simulink model "r2_b8a4x128f_4gbe"  (R2012b)
settings: Solver=VariableStepDiscrete  SolverMode=SingleTasking  StartTime=0.0  StopTime=1  RelTol=1e-3
undefined symbols (not defined in the file): fft_stages, n_ants, n_bits_xengs
libraries: xbsIndex_r4 x21845, casper_library_misc x157, xbsReplacements_r4 x24, casper_library_communications x8, casper_library_delays x8, xps_library x5
(part 58 of 182)

== system r2_b8a4x128f_4gbe/sys3/vacc_tvg ==
  tvg_sel : Inport
  sync_in : Inport  Port=2
  data_in : Inport  Port=3
  valid_in : Inport  Port=4
  misci : Inport  Port=5
  Delay{,1..4} (5 alike) : xbsIndex_r4/Delay  rst=off  infoeditControl=Selection of Reset will increase slice count due to use of real FFs and instead of SRLs  en=off  latency=1  dbl_ovrd=off  reg_retiming=on  block_type=delay
      settings: xl_area=[0, 0, 0, 0, 0, 0, 0]
  Mux1 : xbsIndex_r4/Mux  inputs=2  en=off  latency=0  precision=Full  arith_type="Signed  (2's comp)"  n_bits=8  bin_pt=2  quantization=Truncate  overflow=Wrap  dbl_ovrd=off  block_type=mux
      settings: xl_area=[0, 0, 0, 0, 0, 0, 0]
  Mux2 : xbsIndex_r4/Mux  inputs=2  en=off  latency=0  precision=Full  arith_type="Signed  (2's comp)"  n_bits=8  bin_pt=2  quantization=Truncate  overflow=Wrap  dbl_ovrd=off  block_type=mux
      settings: xl_area=[0, 0, 0, 0, 0, 0, 0]
  Mux3 : xbsIndex_r4/Mux  inputs=2  en=off  latency=0  precision=Full  arith_type="Signed  (2's comp)"  n_bits=8  bin_pt=2  quantization=Truncate  overflow=Wrap  dbl_ovrd=off  block_type=mux
      settings: xl_area=[0, 0, 0, 0, 0, 0, 0]
  Slice : xbsIndex_r4/Slice  nbits=n_bits  boolean_output=off  mode=Lower Bit Location + Width  bit1=0  base1=MSB of Input  bit0=0  base0=LSB of Input  dbl_ovrd=off  block_type=slice
  Slice1 : xbsIndex_r4/Slice  nbits=1  boolean_output=on  mode=Lower Bit Location + Width  bit1=0  base1=MSB of Input  bit0=4  base0=LSB of Input  dbl_ovrd=off  block_type=slice
      settings: infoedit="Extracts a given range of bits from each input sample and presents it at the output.  The output type is ordinarily unsigned with binary point at zero, but can be Boolean when the slice is one bit wide.<P><P>Hardware notes: In hardware this block costs nothing."  block_version=10.1.3
  Slice2 : xbsIndex_r4/Slice  nbits=1  boolean_output=on  mode=Lower Bit Location + Width  bit1=0  base1=MSB of Input  bit0=0  base0=LSB of Input  dbl_ovrd=off  block_type=slice
      settings: infoedit="Extracts a given range of bits from each input sample and presents it at the output.  The output type is ordinarily unsigned with binary point at zero, but can be Boolean when the slice is one bit wide.<P><P>Hardware notes: In hardware this block costs nothing."  block_version=10.1.3
  Slice3 : xbsIndex_r4/Slice  nbits=1  boolean_output=on  mode=Lower Bit Location + Width  bit1=0  base1=MSB of Input  bit0=3  base0=LSB of Input  dbl_ovrd=off  block_type=slice
      settings: infoedit="Extracts a given range of bits from each input sample and presents it at the output.  The output type is ordinarily unsigned with binary point at zero, but can be Boolean when the slice is one bit wide.<P><P>Hardware notes: In hardware this block costs nothing."  block_version=10.1.3
  Slice4 : xbsIndex_r4/Slice  nbits=1  boolean_output=on  mode=Lower Bit Location + Width  bit1=0  base1=MSB of Input  bit0=2  base0=LSB of Input  dbl_ovrd=off  block_type=slice
      settings: infoedit="Extracts a given range of bits from each input sample and presents it at the output.  The output type is ordinarily unsigned with binary point at zero, but can be Boolean when the slice is one bit wide.<P><P>Hardware notes: In hardware this block costs nothing."  block_version=10.1.3
  Slice5 : xbsIndex_r4/Slice  nbits=1  boolean_output=on  mode=Lower Bit Location + Width  bit1=0  base1=MSB of Input  bit0=1  base0=LSB of Input  dbl_ovrd=off  block_type=slice
      settings: infoedit="Extracts a given range of bits from each input sample and presents it at the output.  The output type is ordinarily unsigned with binary point at zero, but can be Boolean when the slice is one bit wide.<P><P>Hardware notes: In hardware this block costs nothing."  block_version=10.1.3
  Slice6 : xbsIndex_r4/Slice  nbits=1  boolean_output=on  mode=Lower Bit Location + Width  bit1=0  base1=MSB of Input  bit0=0  base0=LSB of Input  dbl_ovrd=off  block_type=slice
      settings: infoedit="Extracts a given range of bits from each input sample and presents it at the output.  The output type is ordinarily unsigned with binary point at zero, but can be Boolean when the slice is one bit wide.<P><P>Hardware notes: In hardware this block costs nothing."  block_version=10.1.3
  Slice7 : xbsIndex_r4/Slice  nbits=1  boolean_output=on  mode=Lower Bit Location + Width  bit1=0  base1=MSB of Input  bit0=5  base0=LSB of Input  dbl_ovrd=off  block_type=slice
      settings: infoedit="Extracts a given range of bits from each input sample and presents it at the output.  The output type is ordinarily unsigned with binary point at zero, but can be Boolean when the slice is one bit wide.<P><P>Hardware notes: In hardware this block costs nothing."  block_version=10.1.3
  Slice8 : xbsIndex_r4/Slice  nbits=n_bits  boolean_output=off  mode=Lower Bit Location + Width  bit1=0  base1=MSB of Input  bit0=0  base0=LSB of Input  dbl_ovrd=off  block_type=slice
  Terminator{1..5} (5 alike) : Terminator
  bus_replicate : Subsystem  AncestorBlock=casper_library_bus/bus_replicate  mask(bus_replicate){replication=n_inputs, latency=0, misc=off, implementation=core}
      mask prompts: replication "replication factor"; misc "misc support"; implementation "delay implementation"
      mask help: Output bus formed by replicating input bus a number of times
      mask init:
      | bus_replicate_init(gcb, ...
      |     'replication', replication, ...
      |     'latency', latency, ...
      |     'implementation', implementation, ...
      |     'misc', misc);
      mask TypeOptions implementation: core | behavioral
  bus_replicate1 : Subsystem  AncestorBlock=casper_library_bus/bus_replicate  mask(bus_replicate){replication=n_inputs, latency=0, misc=off, implementation=core}
      mask prompts: replication "replication factor"; misc "misc support"; implementation "delay implementation"
      mask help: Output bus formed by replicating input bus a number of times
      mask init:
      | bus_replicate_init(gcb, ...
      |     'replication', replication, ...
      |     'latency', latency, ...
      |     'implementation', implementation, ...
      |     'misc', misc);
      mask TypeOptions implementation: core | behavioral
  edge_detect : Subsystem  AncestorBlock=casper_library_misc/edge_detect  mask(edge_detect){edge=Rising, polarity=Active High, x_in=[0 0.08 0.08 0.16 0.16 0.24 0.24 0.32 0.32 0.4], y_in=[-1 -1  1  1  1  1  1  1  1  1], x_out=[0.6 0.68 0.68 0.76 0.76 0.84 0.84 0.92 0.92 1], y_out=[-1 -1  1  1 -1 -1 -1 -1 -1 -1]}
      mask prompts: edge "Edge Type"; polarity "Output Polarity"; x_in "Input X Positions"; y_in "Input Y Positions"; x_out "Output X Positions"; y_out "Output Y Positions"
      mask help: Output is active for one-cycle after each edge of the specified type (i.e. rising, falling or both).
      mask init: same as r2_b8a4x128f_4gbe/edge_detect
      settings: AttributesFormatString=|
      | rising edges
      | active high
      mask Help: Output is active for one-cycle after each edge of the specified type (i.e. rising, falling, or both).  Latency is zero.
      mask TypeOptions edge: Rising | Falling | Both
      mask TypeOptions polarity: Active High | Active Low
      mask Display:
      | plot(x_in_num,0.5+y_in_num*0.2);
      | plot(x_out_num,0.5+y_out_num*0.2);
  generate_pulses : Subsystem
  group_period : Subsystem  Tag=xps:sw_reg  AncestorBlock=xps_library/software register  mask(swreg){mode=one value, io_dir=From Processor, io_delay=0, sample_period=1, names=reg, bitwidths=32, arith_types=0, bin_pts=0, show_format=off}
      mask prompts: io_dir "I/O direction"; io_delay "I/O delay"; sample_period "Sample period"; names "Name:"; bitwidths "Bitwidth:"; arith_types "Type (ufix=0, fix=1, bool=2):"; bin_pts "Binary pt:"; show_format "Print format string?"
      mask init:
      | swreg_init(gcb)
      settings: AttributesFormatString=1input
      mask TypeOptions mode: one value | fields of equal size | fields of arbitrary size
      mask Callback mode: swreg_cb(gcb);
      mask TypeOptions io_dir: To Processor | From Processor
      mask Callback io_dir:
      | mask_enables = get_param(gcb, 'MaskEnables');
      | mask_names = get_param(gcb, 'MaskNames');
      | if strcmp(get_param(gcb, 'io_dir'), 'To Processor'),
      |     mask_enables{ismember(mask_names, 'sample_period')} = 'off';
      | else
      |     mask_enables{ismember(mask_names, 'sample_period')} = 'on';
      | end
      | set_param(gcb, 'MaskEnables', mask_enables);
      mask Callback bitwidths:
      | blk = gcb;
      | mode = get_param(blk, 'mode');
      | current_widths = eval(get_param(blk, 'bitwidths'));
      | if (strcmp(mode, 'one value') || strcmp(mode, 'fields of equal size')) && (length(current_widths) > 1),
      |     error('Only one width may be specified for this mode.');
      | elseif strcmp(mode, 'fields of arbitrary size')
      |     current_names = textscan(strtrim(strrep(strrep(get_param(blk, 'names'), ']', ''), '[', '')), '%s');
      |     current_names = current_names{1};
      |     numios = length(current_names);
      |     if length(current_widths) ~= numios,
      |         error('%d field names specified, but %d widths?', numios, length(current_widths));
      |     end
      | end
      | total_width = 0;
      | for ctr = 1 : length(current_widths),
      |     total_width = total_width + current_widths(ctr);
      | end
      | if total_width > 32,
      |     error('Total width must be 32 or less, set to %d.', total_width);
      | end
      mask Callback arith_types:
      | blk = gcb;
      | mode = get_param(blk, 'mode');
      | current_types = eval(get_param(blk, 'arith_types'));
      | numios = length(current_types);
      | if (strcmp(mode, 'one value') || strcmp(mode, 'fields of equal size')) && (length(current_types) > 1),
      |     error('Only one type may be specified for this mode.');
      | elseif strcmp(mode, 'fields of arbitrary size')
      |     current_names = textscan(strtrim(strrep(strrep(get_param(blk, 'names'), ']', ''), '[', '')), '%s');
      |     current_names = current_names{1};
      |     numios = length(current_names);
      |     if length(current_types) ~= numios,
      |         error('%d field names specified, but %d types?', numios, length(current_types));
      |     end
      | end
      | problem = 0;
      | for ctr = 1 : numios,
      |     t = current_types(ctr);
      |     if (t < 0) || (t > 2),
      |         problem = t;
      |         ctr = numios + 1;
      |     end
      | end
      | if problem ~= 0,
      |     error('Type cannot be %i, must be 0, 1 or 2.', problem);
      | end
      mask Callback bin_pts:
      | blk = gcb;
      | mode = get_param(blk, 'mode');
      | current_bins = eval(get_param(blk, 'bin_pts'));
      | if (strcmp(mode, 'one value') || strcmp(mode, 'fields of equal size')) && (length(current_bins) > 1),
      |     error('Only one binary pt may be specified for this mode.');
      | elseif strcmp(mode, 'fields of arbitrary size')
      |     current_names = textscan(strtrim(strrep(strrep(get_param(blk, 'names'), ']', ''), '[', '')), '%s');
      |     current_names = current_names{1};
      |     numios = length(current_names);
      |     if length(current_bins) ~= numios,
      |         error('%d field names specified, but %d binary pts?', numios, length(current_bins));
      |     end
      | end
  ins_counter : Subsystem  mask{vec_len=len/n_inputs, n_inputs=n_inputs, n_bits=n_bits}
      mask prompts: vec_len "Vector Length?"; n_inputs "Simultaneous inputs"; n_bits "Data width"
      mask init:
      | fmtstr = sprintf('Vector Length: %d', vec_len);
      | set_param(gcb, 'AttributesFormatString', fmtstr);
      settings: AttributesFormatString=Vector Length: 9216
  ins_vect_loc : Subsystem  Tag=xps:sw_reg  AncestorBlock=xps_library/software register  mask(swreg){mode=one value, io_dir=From Processor, io_delay=0, sample_period=1, names=reg, bitwidths=32, arith_types=0, bin_pts=0, show_format=off}
      mask prompts: io_dir "I/O direction"; io_delay "I/O delay"; sample_period "Sample period"; names "Name:"; bitwidths "Bitwidth:"; arith_types "Type (ufix=0, fix=1, bool=2):"; bin_pts "Binary pt:"; show_format "Print format string?"
      mask init:
      | swreg_init(gcb)
      settings: AttributesFormatString=1input
      mask TypeOptions mode: one value | fields of equal size | fields of arbitrary size
      mask Callback mode: swreg_cb(gcb);
      mask TypeOptions io_dir: To Processor | From Processor
      mask Callback io_dir:
      | mask_enables = get_param(gcb, 'MaskEnables');
      | mask_names = get_param(gcb, 'MaskNames');
      | if strcmp(get_param(gcb, 'io_dir'), 'To Processor'),
      |     mask_enables{ismember(mask_names, 'sample_period')} = 'off';
      | else
      |     mask_enables{ismember(mask_names, 'sample_period')} = 'on';
      | end
      | set_param(gcb, 'MaskEnables', mask_enables);
      mask Callback bitwidths:
      | blk = gcb;
      | mode = get_param(blk, 'mode');
      | current_widths = eval(get_param(blk, 'bitwidths'));
      | if (strcmp(mode, 'one value') || strcmp(mode, 'fields of equal size')) && (length(current_widths) > 1),
      |     error('Only one width may be specified for this mode.');
      | elseif strcmp(mode, 'fields of arbitrary size')
      |     current_names = textscan(strtrim(strrep(strrep(get_param(blk, 'names'), ']', ''), '[', '')), '%s');
      |     current_names = current_names{1};
      |     numios = length(current_names);
      |     if length(current_widths) ~= numios,
      |         error('%d field names specified, but %d widths?', numios, length(current_widths));
      |     end
      | end
      | total_width = 0;
      | for ctr = 1 : length(current_widths),
      |     total_width = total_width + current_widths(ctr);
      | end
      | if total_width > 32,
      |     error('Total width must be 32 or less, set to %d.', total_width);
      | end
      mask Callback arith_types:
      | blk = gcb;
      | mode = get_param(blk, 'mode');
      | current_types = eval(get_param(blk, 'arith_types'));
      | numios = length(current_types);
      | if (strcmp(mode, 'one value') || strcmp(mode, 'fields of equal size')) && (length(current_types) > 1),
      |     error('Only one type may be specified for this mode.');
      | elseif strcmp(mode, 'fields of arbitrary size')
      |     current_names = textscan(strtrim(strrep(strrep(get_param(blk, 'names'), ']', ''), '[', '')), '%s');
      |     current_names = current_names{1};
      |     numios = length(current_names);
      |     if length(current_types) ~= numios,
      |         error('%d field names specified, but %d types?', numios, length(current_types));
      |     end
      | end
      | problem = 0;
      | for ctr = 1 : numios,
      |     t = current_types(ctr);
      |     if (t < 0) || (t > 2),
      |         problem = t;
      |         ctr = numios + 1;
      |     end
      | end
      | if problem ~= 0,
      |     error('Type cannot be %i, must be 0, 1 or 2.', problem);
      | end
      mask Callback bin_pts:
      | blk = gcb;
      | mode = get_param(blk, 'mode');
      | current_bins = eval(get_param(blk, 'bin_pts'));
      | if (strcmp(mode, 'one value') || strcmp(mode, 'fields of equal size')) && (length(current_bins) > 1),
      |     error('Only one binary pt may be specified for this mode.');
      | elseif strcmp(mode, 'fields of arbitrary size')
      |     current_names = textscan(strtrim(strrep(strrep(get_param(blk, 'names'), ']', ''), '[', '')), '%s');
      |     current_names = current_names{1};
      |     numios = length(current_names);
      |     if length(current_bins) ~= numios,
      |         error('%d field names specified, but %d binary pts?', numios, length(current_bins));
      |     end
      | end
  ins_vect_val : Subsystem  Tag=xps:sw_reg  AncestorBlock=xps_library/software register  mask(swreg){mode=one value, io_dir=From Processor, io_delay=0, sample_period=1, names=reg, bitwidths=32, arith_types=0, bin_pts=0, show_format=off}
      mask prompts: io_dir "I/O direction"; io_delay "I/O delay"; sample_period "Sample period"; names "Name:"; bitwidths "Bitwidth:"; arith_types "Type (ufix=0, fix=1, bool=2):"; bin_pts "Binary pt:"; show_format "Print format string?"
      mask init:
      | swreg_init(gcb)
      settings: AttributesFormatString=1input
      mask TypeOptions mode: one value | fields of equal size | fields of arbitrary size
      mask Callback mode: swreg_cb(gcb);
      mask TypeOptions io_dir: To Processor | From Processor
      mask Callback io_dir:
      | mask_enables = get_param(gcb, 'MaskEnables');
      | mask_names = get_param(gcb, 'MaskNames');
      | if strcmp(get_param(gcb, 'io_dir'), 'To Processor'),
      |     mask_enables{ismember(mask_names, 'sample_period')} = 'off';
      | else
      |     mask_enables{ismember(mask_names, 'sample_period')} = 'on';
      | end
      | set_param(gcb, 'MaskEnables', mask_enables);
      mask Callback bitwidths:
      | blk = gcb;
      | mode = get_param(blk, 'mode');
      | current_widths = eval(get_param(blk, 'bitwidths'));
      | if (strcmp(mode, 'one value') || strcmp(mode, 'fields of equal size')) && (length(current_widths) > 1),
      |     error('Only one width may be specified for this mode.');
      | elseif strcmp(mode, 'fields of arbitrary size')
      |     current_names = textscan(strtrim(strrep(strrep(get_param(blk, 'names'), ']', ''), '[', '')), '%s');
      |     current_names = current_names{1};
      |     numios = length(current_names);
      |     if length(current_widths) ~= numios,
      |         error('%d field names specified, but %d widths?', numios, length(current_widths));
      |     end
      | end
      | total_width = 0;
      | for ctr = 1 : length(current_widths),
      |     total_width = total_width + current_widths(ctr);
      | end
      | if total_width > 32,
      |     error('Total width must be 32 or less, set to %d.', total_width);
      | end
      mask Callback arith_types:
      | blk = gcb;
      | mode = get_param(blk, 'mode');
      | current_types = eval(get_param(blk, 'arith_types'));
      | numios = length(current_types);
      | if (strcmp(mode, 'one value') || strcmp(mode, 'fields of equal size')) && (length(current_types) > 1),
      |     error('Only one type may be specified for this mode.');
      | elseif strcmp(mode, 'fields of arbitrary size')
      |     current_names = textscan(strtrim(strrep(strrep(get_param(blk, 'names'), ']', ''), '[', '')), '%s');
      |     current_names = current_names{1};
      |     numios = length(current_names);
      |     if length(current_types) ~= numios,
      |         error('%d field names specified, but %d types?', numios, length(current_types));
      |     end
      | end
      | problem = 0;
      | for ctr = 1 : numios,
      |     t = current_types(ctr);
      |     if (t < 0) || (t > 2),
      |         problem = t;
      |         ctr = numios + 1;
      |     end
      | end
      | if problem ~= 0,
      |     error('Type cannot be %i, must be 0, 1 or 2.', problem);
      | end
      mask Callback bin_pts:
      | blk = gcb;
      | mode = get_param(blk, 'mode');
      | current_bins = eval(get_param(blk, 'bin_pts'));
      | if (strcmp(mode, 'one value') || strcmp(mode, 'fields of equal size')) && (length(current_bins) > 1),
      |     error('Only one binary pt may be specified for this mode.');
      | elseif strcmp(mode, 'fields of arbitrary size')
      |     current_names = textscan(strtrim(strrep(strrep(get_param(blk, 'names'), ']', ''), '[', '')), '%s');
      |     current_names = current_names{1};
      |     numios = length(current_names);
      |     if length(current_bins) ~= numios,
      |         error('%d field names specified, but %d binary pts?', numios, length(current_bins));
      |     end
      | end
  ins_vector : Subsystem  mask{num_vectors=len/n_inputs}
      mask prompts: num_vectors "number of vectors"
      mask init:
      | fmtstr = sprintf('Vector Length: %d', num_vectors);
      | set_param(gcb, 'AttributesFormatString', fmtstr);
      settings: AttributesFormatString=Vector Length: 9216
  master_reset_sim1 : Constant  Value=0
  master_reset_sim10 : Constant  Value=1000
  master_reset_sim11 : Constant  Value=127
  master_reset_sim4 : Constant  Value=0
  master_reset_sim7 : Constant  Value=512000
  master_reset_sim8 : Constant
  master_reset_sim9 : Constant  Value=3
  n_per_group : Subsystem  Tag=xps:sw_reg  AncestorBlock=xps_library/software register  mask(swreg){mode=one value, io_dir=From Processor, io_delay=0, sample_period=1, names=reg, bitwidths=32, arith_types=0, bin_pts=0, show_format=off}
      mask prompts: io_dir "I/O direction"; io_delay "I/O delay"; sample_period "Sample period"; names "Name:"; bitwidths "Bitwidth:"; arith_types "Type (ufix=0, fix=1, bool=2):"; bin_pts "Binary pt:"; show_format "Print format string?"
      mask init:
      | swreg_init(gcb)
      settings: AttributesFormatString=1input
      mask TypeOptions mode: one value | fields of equal size | fields of arbitrary size
      mask Callback mode: swreg_cb(gcb);
      mask TypeOptions io_dir: To Processor | From Processor
      mask Callback io_dir:
      | mask_enables = get_param(gcb, 'MaskEnables');
      | mask_names = get_param(gcb, 'MaskNames');
      | if strcmp(get_param(gcb, 'io_dir'), 'To Processor'),
      |     mask_enables{ismember(mask_names, 'sample_period')} = 'off';
      | else
      |     mask_enables{ismember(mask_names, 'sample_period')} = 'on';
      | end
      | set_param(gcb, 'MaskEnables', mask_enables);
      mask Callback bitwidths:
      | blk = gcb;
      | mode = get_param(blk, 'mode');
      | current_widths = eval(get_param(blk, 'bitwidths'));
      | if (strcmp(mode, 'one value') || strcmp(mode, 'fields of equal size')) && (length(current_widths) > 1),
      |     error('Only one width may be specified for this mode.');
      | elseif strcmp(mode, 'fields of arbitrary size')
      |     current_names = textscan(strtrim(strrep(strrep(get_param(blk, 'names'), ']', ''), '[', '')), '%s');
      |     current_names = current_names{1};
      |     numios = length(current_names);
      |     if length(current_widths) ~= numios,
      |         error('%d field names specified, but %d widths?', numios, length(current_widths));
      |     end
      | end
      | total_width = 0;
      | for ctr = 1 : length(current_widths),
      |     total_width = total_width + current_widths(ctr);
      | end
      | if total_width > 32,
      |     error('Total width must be 32 or less, set to %d.', total_width);
      | end
      mask Callback arith_types:
      | blk = gcb;
      | mode = get_param(blk, 'mode');
      | current_types = eval(get_param(blk, 'arith_types'));
      | numios = length(current_types);
      | if (strcmp(mode, 'one value') || strcmp(mode, 'fields of equal size')) && (length(current_types) > 1),
      |     error('Only one type may be specified for this mode.');
      | elseif strcmp(mode, 'fields of arbitrary size')
      |     current_names = textscan(strtrim(strrep(strrep(get_param(blk, 'names'), ']', ''), '[', '')), '%s');
      |     current_names = current_names{1};
      |     numios = length(current_names);
      |     if length(current_types) ~= numios,
      |         error('%d field names specified, but %d types?', numios, length(current_types));
      |     end
      | end
      | problem = 0;
      | for ctr = 1 : numios,
      |     t = current_types(ctr);
      |     if (t < 0) || (t > 2),
      |         problem = t;
      |         ctr = numios + 1;
      |     end
      | end
      | if problem ~= 0,
      |     error('Type cannot be %i, must be 0, 1 or 2.', problem);
      | end
      mask Callback bin_pts:
      | blk = gcb;
      | mode = get_param(blk, 'mode');
      | current_bins = eval(get_param(blk, 'bin_pts'));
      | if (strcmp(mode, 'one value') || strcmp(mode, 'fields of equal size')) && (length(current_bins) > 1),
      |     error('Only one binary pt may be specified for this mode.');
      | elseif strcmp(mode, 'fields of arbitrary size')
      |     current_names = textscan(strtrim(strrep(strrep(get_param(blk, 'names'), ']', ''), '[', '')), '%s');
      |     current_names = current_names{1};
      |     numios = length(current_names);
      |     if length(current_bins) ~= numios,
      |         error('%d field names specified, but %d binary pts?', numios, length(current_bins));
      |     end
      | end
  n_pulses : Subsystem  Tag=xps:sw_reg  AncestorBlock=xps_library/software register  mask(swreg){mode=one value, io_dir=From Processor, io_delay=0, sample_period=1, names=reg, bitwidths=32, arith_types=0, bin_pts=0, show_format=off}
      mask prompts: io_dir "I/O direction"; io_delay "I/O delay"; sample_period "Sample period"; names "Name:"; bitwidths "Bitwidth:"; arith_types "Type (ufix=0, fix=1, bool=2):"; bin_pts "Binary pt:"; show_format "Print format string?"
      mask init:
      | swreg_init(gcb)
      settings: AttributesFormatString=1input
      mask TypeOptions mode: one value | fields of equal size | fields of arbitrary size
      mask Callback mode: swreg_cb(gcb);
      mask TypeOptions io_dir: To Processor | From Processor
      mask Callback io_dir:
      | mask_enables = get_param(gcb, 'MaskEnables');
      | mask_names = get_param(gcb, 'MaskNames');
      | if strcmp(get_param(gcb, 'io_dir'), 'To Processor'),
      |     mask_enables{ismember(mask_names, 'sample_period')} = 'off';
      | else
      |     mask_enables{ismember(mask_names, 'sample_period')} = 'on';
      | end
      | set_param(gcb, 'MaskEnables', mask_enables);
      mask Callback bitwidths:
      | blk = gcb;
      | mode = get_param(blk, 'mode');
      | current_widths = eval(get_param(blk, 'bitwidths'));
      | if (strcmp(mode, 'one value') || strcmp(mode, 'fields of equal size')) && (length(current_widths) > 1),
      |     error('Only one width may be specified for this mode.');
      | elseif strcmp(mode, 'fields of arbitrary size')
      |     current_names = textscan(strtrim(strrep(strrep(get_param(blk, 'names'), ']', ''), '[', '')), '%s');
      |     current_names = current_names{1};
      |     numios = length(current_names);
      |     if length(current_widths) ~= numios,
      |         error('%d field names specified, but %d widths?', numios, length(current_widths));
      |     end
      | end
      | total_width = 0;
      | for ctr = 1 : length(current_widths),
      |     total_width = total_width + current_widths(ctr);
      | end
      | if total_width > 32,
      |     error('Total width must be 32 or less, set to %d.', total_width);
      | end
      mask Callback arith_types:
      | blk = gcb;
      | mode = get_param(blk, 'mode');
      | current_types = eval(get_param(blk, 'arith_types'));
      | numios = length(current_types);
      | if (strcmp(mode, 'one value') || strcmp(mode, 'fields of equal size')) && (length(current_types) > 1),
      |     error('Only one type may be specified for this mode.');
      | elseif strcmp(mode, 'fields of arbitrary size')
      |     current_names = textscan(strtrim(strrep(strrep(get_param(blk, 'names'), ']', ''), '[', '')), '%s');
      |     current_names = current_names{1};
      |     numios = length(current_names);
      |     if length(current_types) ~= numios,
      |         error('%d field names specified, but %d types?', numios, length(current_types));
      |     end
      | end
      | problem = 0;
      | for ctr = 1 : numios,
      |     t = current_types(ctr);
      |     if (t < 0) || (t > 2),
      |         problem = t;
      |         ctr = numios + 1;
      |     end
      | end
      | if problem ~= 0,
      |     error('Type cannot be %i, must be 0, 1 or 2.', problem);
      | end
      mask Callback bin_pts:
      | blk = gcb;
      | mode = get_param(blk, 'mode');
      | current_bins = eval(get_param(blk, 'bin_pts'));
      | if (strcmp(mode, 'one value') || strcmp(mode, 'fields of equal size')) && (length(current_bins) > 1),
      |     error('Only one binary pt may be specified for this mode.');
      | elseif strcmp(mode, 'fields of arbitrary size')
      |     current_names = textscan(strtrim(strrep(strrep(get_param(blk, 'names'), ']', ''), '[', '')), '%s');
      |     current_names = current_names{1};
      |     numios = length(current_names);
      |     if length(current_bins) ~= numios,
      |         error('%d field names specified, but %d binary pts?', numios, length(current_bins));
      |     end
      | end
  reset_vbs : Subsystem  Tag=xps:sw_reg  AncestorBlock=xps_library/software register  mask(swreg){mode=one value, io_dir=From Processor, io_delay=0, sample_period=1, names=reg, bitwidths=32, arith_types=0, bin_pts=0, show_format=off}
      mask prompts: io_dir "I/O direction"; io_delay "I/O delay"; sample_period "Sample period"; names "Name:"; bitwidths "Bitwidth:"; arith_types "Type (ufix=0, fix=1, bool=2):"; bin_pts "Binary pt:"; show_format "Print format string?"
      mask init:
      | swreg_init(gcb)
      settings: AttributesFormatString=1input
      mask TypeOptions mode: one value | fields of equal size | fields of arbitrary size
      mask Callback mode: swreg_cb(gcb);
      mask TypeOptions io_dir: To Processor | From Processor
      mask Callback io_dir:
      | mask_enables = get_param(gcb, 'MaskEnables');
      | mask_names = get_param(gcb, 'MaskNames');
      | if strcmp(get_param(gcb, 'io_dir'), 'To Processor'),
      |     mask_enables{ismember(mask_names, 'sample_period')} = 'off';
      | else
      |     mask_enables{ismember(mask_names, 'sample_period')} = 'on';
      | end
      | set_param(gcb, 'MaskEnables', mask_enables);
      mask Callback bitwidths:
      | blk = gcb;
      | mode = get_param(blk, 'mode');
      | current_widths = eval(get_param(blk, 'bitwidths'));
      | if (strcmp(mode, 'one value') || strcmp(mode, 'fields of equal size')) && (length(current_widths) > 1),
      |     error('Only one width may be specified for this mode.');
      | elseif strcmp(mode, 'fields of arbitrary size')
      |     current_names = textscan(strtrim(strrep(strrep(get_param(blk, 'names'), ']', ''), '[', '')), '%s');
      |     current_names = current_names{1};
      |     numios = length(current_names);
      |     if length(current_widths) ~= numios,
      |         error('%d field names specified, but %d widths?', numios, length(current_widths));
      |     end
      | end
      | total_width = 0;
      | for ctr = 1 : length(current_widths),
      |     total_width = total_width + current_widths(ctr);
      | end
      | if total_width > 32,
      |     error('Total width must be 32 or less, set to %d.', total_width);
      | end
      mask Callback arith_types:
      | blk = gcb;
      | mode = get_param(blk, 'mode');
      | current_types = eval(get_param(blk, 'arith_types'));
      | numios = length(current_types);
      | if (strcmp(mode, 'one value') || strcmp(mode, 'fields of equal size')) && (length(current_types) > 1),
      |     error('Only one type may be specified for this mode.');
      | elseif strcmp(mode, 'fields of arbitrary size')
      |     current_names = textscan(strtrim(strrep(strrep(get_param(blk, 'names'), ']', ''), '[', '')), '%s');
      |     current_names = current_names{1};
      |     numios = length(current_names);
      |     if length(current_types) ~= numios,
      |         error('%d field names specified, but %d types?', numios, length(current_types));
      |     end
      | end
      | problem = 0;
      | for ctr = 1 : numios,
      |     t = current_types(ctr);
      |     if (t < 0) || (t > 2),
      |         problem = t;
      |         ctr = numios + 1;
      |     end
      | end
      | if problem ~= 0,
      |     error('Type cannot be %i, must be 0, 1 or 2.', problem);
      | end
      mask Callback bin_pts:
      | blk = gcb;
      | mode = get_param(blk, 'mode');
      | current_bins = eval(get_param(blk, 'bin_pts'));
      | if (strcmp(mode, 'one value') || strcmp(mode, 'fields of equal size')) && (length(current_bins) > 1),
      |     error('Only one binary pt may be specified for this mode.');
      | elseif strcmp(mode, 'fields of arbitrary size')
      |     current_names = textscan(strtrim(strrep(strrep(get_param(blk, 'names'), ']', ''), '[', '')), '%s');
      |     current_names = current_names{1};
      |     numios = length(current_names);
      |     if length(current_bins) ~= numios,
      |         error('%d field names specified, but %d binary pts?', numios, length(current_bins));
      |     end
      | end
  valid_bet_sync : Subsystem
  valid_bet_sync_sync : Subsystem
  vbs_dram : Subsystem  Tag=xps:sw_reg  AncestorBlock=xps_library/software register  mask(swreg){mode=one value, io_dir=To Processor, io_delay=0, sample_period=1, names=reg, bitwidths=32, arith_types=0, bin_pts=0, show_format=off}
      mask prompts: io_dir "I/O direction"; io_delay "I/O delay"; sample_period "Sample period"; names "Name:"; bitwidths "Bitwidth:"; arith_types "Type (ufix=0, fix=1, bool=2):"; bin_pts "Binary pt:"; show_format "Print format string?"
      mask init:
      | swreg_init(gcb)
      settings: AttributesFormatString=1output
      mask TypeOptions mode: one value | fields of equal size | fields of arbitrary size
      mask Callback mode: swreg_cb(gcb);
      mask TypeOptions io_dir: To Processor | From Processor
      mask Callback io_dir:
      | mask_enables = get_param(gcb, 'MaskEnables');
      | mask_names = get_param(gcb, 'MaskNames');
      | if strcmp(get_param(gcb, 'io_dir'), 'To Processor'),
      |     mask_enables{ismember(mask_names, 'sample_period')} = 'off';
      | else
      |     mask_enables{ismember(mask_names, 'sample_period')} = 'on';
      | end
      | set_param(gcb, 'MaskEnables', mask_enables);
      mask Callback bitwidths:
      | blk = gcb;
      | mode = get_param(blk, 'mode');
      | current_widths = eval(get_param(blk, 'bitwidths'));
      | if (strcmp(mode, 'one value') || strcmp(mode, 'fields of equal size')) && (length(current_widths) > 1),
      |     error('Only one width may be specified for this mode.');
      | elseif strcmp(mode, 'fields of arbitrary size')
      |     current_names = textscan(strtrim(strrep(strrep(get_param(blk, 'names'), ']', ''), '[', '')), '%s');
      |     current_names = current_names{1};
      |     numios = length(current_names);
      |     if length(current_widths) ~= numios,
      |         error('%d field names specified, but %d widths?', numios, length(current_widths));
      |     end
      | end
      | total_width = 0;
      | for ctr = 1 : length(current_widths),
      |     total_width = total_width + current_widths(ctr);
      | end
      | if total_width > 32,
      |     error('Total width must be 32 or less, set to %d.', total_width);
      | end
      mask Callback arith_types:
      | blk = gcb;
      | mode = get_param(blk, 'mode');
      | current_types = eval(get_param(blk, 'arith_types'));
      | numios = length(current_types);
      | if (strcmp(mode, 'one value') || strcmp(mode, 'fields of equal size')) && (length(current_types) > 1),
      |     error('Only one type may be specified for this mode.');
      | elseif strcmp(mode, 'fields of arbitrary size')
      |     current_names = textscan(strtrim(strrep(strrep(get_param(blk, 'names'), ']', ''), '[', '')), '%s');
      |     current_names = current_names{1};
      |     numios = length(current_names);
      |     if length(current_types) ~= numios,
      |         error('%d field names specified, but %d types?', numios, length(current_types));
      |     end
      | end
      | problem = 0;
      | for ctr = 1 : numios,
      |     t = current_types(ctr);
      |     if (t < 0) || (t > 2),
      |         problem = t;
      |         ctr = numios + 1;
      |     end
      | end
      | if problem ~= 0,
      |     error('Type cannot be %i, must be 0, 1 or 2.', problem);
      | end
      mask Callback bin_pts:
      | blk = gcb;
      | mode = get_param(blk, 'mode');
      | current_bins = eval(get_param(blk, 'bin_pts'));
      | if (strcmp(mode, 'one value') || strcmp(mode, 'fields of equal size')) && (length(current_bins) > 1),
      |     error('Only one binary pt may be specified for this mode.');
      | elseif strcmp(mode, 'fields of arbitrary size')
      |     current_names = textscan(strtrim(strrep(strrep(get_param(blk, 'names'), ']', ''), '[', '')), '%s');
      |     current_names = current_names{1};
      |     numios = length(current_names);
      |     if length(current_bins) ~= numios,
      |         error('%d field names specified, but %d binary pts?', numios, length(current_bins));
      |     end
      | end
  vbs_gen : Subsystem  Tag=xps:sw_reg  AncestorBlock=xps_library/software register  mask(swreg){mode=one value, io_dir=To Processor, io_delay=0, sample_period=1, names=reg, bitwidths=32, arith_types=0, bin_pts=0, show_format=off}
      mask prompts: io_dir "I/O direction"; io_delay "I/O delay"; sample_period "Sample period"; names "Name:"; bitwidths "Bitwidth:"; arith_types "Type (ufix=0, fix=1, bool=2):"; bin_pts "Binary pt:"; show_format "Print format string?"
      mask init:
      | swreg_init(gcb)
      settings: AttributesFormatString=1output
      mask TypeOptions mode: one value | fields of equal size | fields of arbitrary size
      mask Callback mode: swreg_cb(gcb);
      mask TypeOptions io_dir: To Processor | From Processor
      mask Callback io_dir:
      | mask_enables = get_param(gcb, 'MaskEnables');
      | mask_names = get_param(gcb, 'MaskNames');
      | if strcmp(get_param(gcb, 'io_dir'), 'To Processor'),
      |     mask_enables{ismember(mask_names, 'sample_period')} = 'off';
      | else
      |     mask_enables{ismember(mask_names, 'sample_period')} = 'on';
      | end
      | set_param(gcb, 'MaskEnables', mask_enables);
      mask Callback bitwidths:
      | blk = gcb;
      | mode = get_param(blk, 'mode');
      | current_widths = eval(get_param(blk, 'bitwidths'));
      | if (strcmp(mode, 'one value') || strcmp(mode, 'fields of equal size')) && (length(current_widths) > 1),
      |     error('Only one width may be specified for this mode.');
      | elseif strcmp(mode, 'fields of arbitrary size')
      |     current_names = textscan(strtrim(strrep(strrep(get_param(blk, 'names'), ']', ''), '[', '')), '%s');
      |     current_names = current_names{1};
      |     numios = length(current_names);
      |     if length(current_widths) ~= numios,
      |         error('%d field names specified, but %d widths?', numios, length(current_widths));
      |     end
      | end
      | total_width = 0;
      | for ctr = 1 : length(current_widths),
      |     total_width = total_width + current_widths(ctr);
      | end
      | if total_width > 32,
      |     error('Total width must be 32 or less, set to %d.', total_width);
      | end
      mask Callback arith_types:
      | blk = gcb;
      | mode = get_param(blk, 'mode');
      | current_types = eval(get_param(blk, 'arith_types'));
      | numios = length(current_types);
      | if (strcmp(mode, 'one value') || strcmp(mode, 'fields of equal size')) && (length(current_types) > 1),
      |     error('Only one type may be specified for this mode.');
      | elseif strcmp(mode, 'fields of arbitrary size')
      |     current_names = textscan(strtrim(strrep(strrep(get_param(blk, 'names'), ']', ''), '[', '')), '%s');
      |     current_names = current_names{1};
      |     numios = length(current_names);
      |     if length(current_types) ~= numios,
      |         error('%d field names specified, but %d types?', numios, length(current_types));
      |     end
      | end
      | problem = 0;
      | for ctr = 1 : numios,
      |     t = current_types(ctr);
      |     if (t < 0) || (t > 2),
      |         problem = t;
      |         ctr = numios + 1;
      |     end
      | end
      | if problem ~= 0,
      |     error('Type cannot be %i, must be 0, 1 or 2.', problem);
      | end
      mask Callback bin_pts:
      | blk = gcb;
      | mode = get_param(blk, 'mode');
      | current_bins = eval(get_param(blk, 'bin_pts'));
      | if (strcmp(mode, 'one value') || strcmp(mode, 'fields of equal size')) && (length(current_bins) > 1),
      |     error('Only one binary pt may be specified for this mode.');
      | elseif strcmp(mode, 'fields of arbitrary size')
      |     current_names = textscan(strtrim(strrep(strrep(get_param(blk, 'names'), ']', ''), '[', '')), '%s');
      |     current_names = current_names{1};
      |     numios = length(current_names);
      |     if length(current_bins) ~= numios,
      |         error('%d field names specified, but %d binary pts?', numios, length(current_bins));
      |     end
      | end
  write : Subsystem  Tag=xps:sw_reg  AncestorBlock=xps_library/software register  mask(swreg){mode=one value, io_dir=From Processor, io_delay=0, sample_period=1, names=reg, bitwidths=32, arith_types=0, bin_pts=0, show_format=off}
      mask prompts: io_dir "I/O direction"; io_delay "I/O delay"; sample_period "Sample period"; names "Name:"; bitwidths "Bitwidth:"; arith_types "Type (ufix=0, fix=1, bool=2):"; bin_pts "Binary pt:"; show_format "Print format string?"
      mask init:
      | swreg_init(gcb)
      settings: AttributesFormatString=1input
      mask TypeOptions mode: one value | fields of equal size | fields of arbitrary size
      mask Callback mode: swreg_cb(gcb);
      mask TypeOptions io_dir: To Processor | From Processor
      mask Callback io_dir:
      | mask_enables = get_param(gcb, 'MaskEnables');
      | mask_names = get_param(gcb, 'MaskNames');
      | if strcmp(get_param(gcb, 'io_dir'), 'To Processor'),
      |     mask_enables{ismember(mask_names, 'sample_period')} = 'off';
      | else
      |     mask_enables{ismember(mask_names, 'sample_period')} = 'on';
      | end
      | set_param(gcb, 'MaskEnables', mask_enables);
      mask Callback bitwidths:
      | blk = gcb;
      | mode = get_param(blk, 'mode');
      | current_widths = eval(get_param(blk, 'bitwidths'));
      | if (strcmp(mode, 'one value') || strcmp(mode, 'fields of equal size')) && (length(current_widths) > 1),
      |     error('Only one width may be specified for this mode.');
      | elseif strcmp(mode, 'fields of arbitrary size')
      |     current_names = textscan(strtrim(strrep(strrep(get_param(blk, 'names'), ']', ''), '[', '')), '%s');
      |     current_names = current_names{1};
      |     numios = length(current_names);
      |     if length(current_widths) ~= numios,
      |         error('%d field names specified, but %d widths?', numios, length(current_widths));
      |     end
      | end
      | total_width = 0;
      | for ctr = 1 : length(current_widths),
      |     total_width = total_width + current_widths(ctr);
      | end
      | if total_width > 32,
      |     error('Total width must be 32 or less, set to %d.', total_width);
      | end
      mask Callback arith_types:
      | blk = gcb;
      | mode = get_param(blk, 'mode');
      | current_types = eval(get_param(blk, 'arith_types'));
      | numios = length(current_types);
      | if (strcmp(mode, 'one value') || strcmp(mode, 'fields of equal size')) && (length(current_types) > 1),
      |     error('Only one type may be specified for this mode.');
      | elseif strcmp(mode, 'fields of arbitrary size')
      |     current_names = textscan(strtrim(strrep(strrep(get_param(blk, 'names'), ']', ''), '[', '')), '%s');
      |     current_names = current_names{1};
      |     numios = length(current_names);
      |     if length(current_types) ~= numios,
      |         error('%d field names specified, but %d types?', numios, length(current_types));
      |     end
      | end
      | problem = 0;
      | for ctr = 1 : numios,
      |     t = current_types(ctr);
      |     if (t < 0) || (t > 2),
      |         problem = t;
      |         ctr = numios + 1;
      |     end
      | end
      | if problem ~= 0,
      |     error('Type cannot be %i, must be 0, 1 or 2.', problem);
      | end
      mask Callback bin_pts:
      | blk = gcb;
      | mode = get_param(blk, 'mode');
      | current_bins = eval(get_param(blk, 'bin_pts'));
      | if (strcmp(mode, 'one value') || strcmp(mode, 'fields of equal size')) && (length(current_bins) > 1),
      |     error('Only one binary pt may be specified for this mode.');
      | elseif strcmp(mode, 'fields of arbitrary size')
      |     current_names = textscan(strtrim(strrep(strrep(get_param(blk, 'names'), ']', ''), '[', '')), '%s');
      |     current_names = current_names{1};
      |     numios = length(current_names);
      |     if length(current_bins) ~= numios,
      |         error('%d field names specified, but %d binary pts?', numios, length(current_bins));
      |     end
      | end
  sync_out : Outport
  data_out : Outport  Port=2
  valid_out : Outport  Port=3
  misco : Outport  Port=4
  wires:
  ins_vector/4(misco) -> misco/1
  ins_counter/4(misco) -> ins_vector/7(misci)
  misci/1 -> ins_counter/5(misci)
  bus_replicate1/1(out) -> Mux2/3
  Slice8/1 -> bus_replicate1/1(in)
  bus_replicate/1(out) -> ins_vector/5(value)
  Slice/1 -> bus_replicate/1(in)
  generate_pulses/2(running) -> Terminator5/1
  vbs_dram/1(sim_out) -> Terminator4/1
  vbs_gen/1(sim_out) -> Terminator3/1
  valid_bet_sync_sync/2(count) -> Terminator1/1
  valid_bet_sync/2(count) -> Terminator2/1
  Delay/1 -> generate_pulses/1(run)
  valid_bet_sync_sync/1(max_count) -> vbs_dram/1(out_reg)
  reset_vbs/1(in_reg) -> Slice2/1
  Slice2/1 -> valid_bet_sync_sync/2(rst_max), valid_bet_sync/2(rst_max)
  master_reset_sim4/1 -> reset_vbs/1(sim_1)
  valid_bet_sync/1(max_count) -> vbs_gen/1(out_reg)
  Slice7/1 -> [rst]
  Slice6/1 -> [enable]
  [inj_counter] -> ins_counter/4(enable)
  ins_vect_val/1(in_reg) -> Slice/1
  master_reset_sim10/1 -> ins_vect_val/1(sim_1)
  ins_vect_loc/1(in_reg) -> ins_vector/4(vector)
  master_reset_sim11/1 -> ins_vect_loc/1(sim_1)
  [inj_vector] -> ins_vector/6(enable)
  edge_detect/1(out) -> valid_bet_sync/1(sync), Mux3/3
  generate_pulses/1(valid) -> Delay1/1
  ins_counter/3(valid_out) -> ins_vector/3(valid_in)
  ins_counter/2(dout) -> ins_vector/2(data_in)
  [enable] -> Delay/1
  Slice1/1 -> [inj_counter]
  Slice3/1 -> [inj_vector]
  [valid_sel] -> Mux1/1
  [data_sel] -> Mux2/1
  [valid_sel] -> Mux3/1
  Slice4/1 -> [valid_sel]
  tvg_sel/1 -> Slice7/1, Slice1/1, Slice3/1, Slice4/1, Slice5/1, Slice6/1
  Slice5/1 -> [data_sel]
  Mux3/1 -> ins_counter/1(new_acc_in)
  sync_in/1 -> Mux3/2
  data_in/1 -> Mux2/2
  Mux2/1 -> ins_counter/2(din)
  ins_counter/1(new_acc_out) -> ins_vector/1(new_acc_in)
  ins_vector/3(valid_out) -> valid_out/1, valid_bet_sync_sync/3(valid)
  ins_vector/2(data) -> data_out/1
  ins_vector/1(new_acc_out) -> valid_bet_sync_sync/1(sync), sync_out/1
  valid_in/1 -> Mux1/2
  Mux1/1 -> ins_counter/3(valid_in)
  master_reset_sim9/1 -> group_period/1(sim_1)
  group_period/1(in_reg) -> Delay4/1
  master_reset_sim8/1 -> n_per_group/1(sim_1)
  n_per_group/1(in_reg) -> Delay3/1
  master_reset_sim7/1 -> n_pulses/1(sim_1)
  n_pulses/1(in_reg) -> Delay2/1
  [rst] -> edge_detect/1(in)
  master_reset_sim1/1 -> write/1(sim_1)
  write/1(in_reg) -> Slice8/1
  Delay1/1 -> valid_bet_sync/3(valid), Mux1/3
  Delay2/1 -> generate_pulses/2(num_pulses)
  Delay3/1 -> generate_pulses/3(num_per_group)
  Delay4/1 -> generate_pulses/4(group period)
